simulink model "task4_simulink"  (R2026a)
settings: Solver=VariableStepAuto  StopTime=2
values from neighbouring files (symbols this model uses):
  K = place(A, B, desired_poles)    [task3.m]    (also in task4.m; task5.m; task5_original.m)
  x0 = initial_conditions(i,:)'    [task4.m]    (also in task5.m = [0; task5_original.m = [0)
settings Model: Creator=DELL  LastModifiedBy=DELL

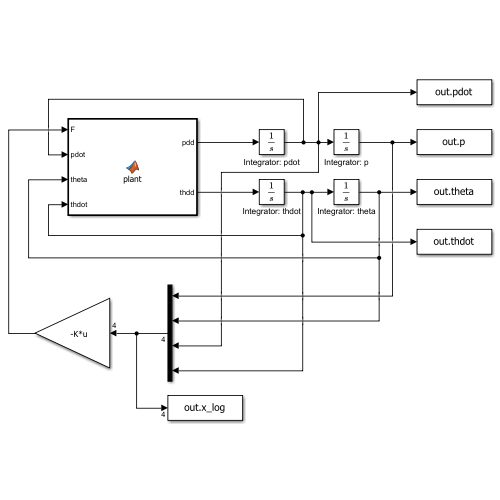
[thumbnail: Simulink's stored preview of the top-level diagram]
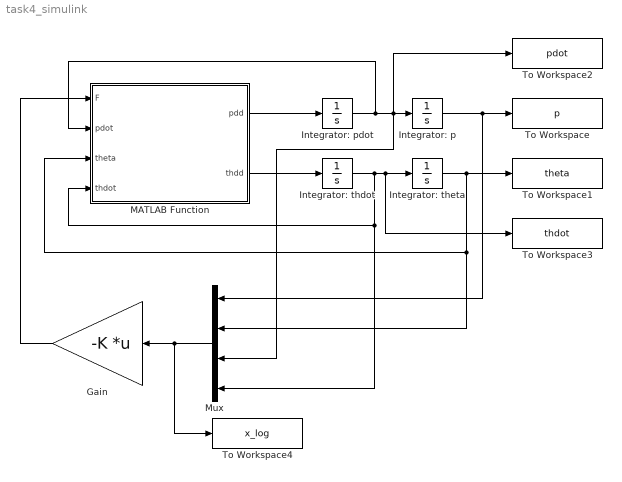
== system task4_simulink ==
  Gain : Gain  Gain=-K  Multiplication=Matrix(K*u)
  Integrator: p : Integrator  InitialCondition=x0(1)
  Integrator: pdot : Integrator  InitialCondition=x0(3)
  Integrator: thdot : Integrator  InitialCondition=x0(4)
  Integrator: theta : Integrator  InitialCondition=x0(2)
  MATLAB Function : MATLAB Function  TreatAsAtomicUnit=on
  Mux : Mux
  To Workspace : ToWorkspace  VariableName=p  SaveFormat=Timeseries  SampleTime=0.01
  To Workspace1 : ToWorkspace  VariableName=theta  SaveFormat=Timeseries  SampleTime=0.01
  To Workspace2 : ToWorkspace  VariableName=pdot  SaveFormat=Timeseries  SampleTime=-1
  To Workspace3 : ToWorkspace  VariableName=thdot  SaveFormat=Timeseries  SampleTime=-1
  To Workspace4 : ToWorkspace  VariableName=x_log  SaveFormat=Timeseries  SampleTime=0.01
  wires:
  MATLAB Function/1(pdd) -> Integrator: pdot/1
  MATLAB Function/2(thdd) -> Integrator: thdot/1
  Integrator: pdot/1 -> MATLAB Function/2(pdot), To Workspace2/1, Integrator: p/1, Mux/3
  Integrator: thdot/1 -> Mux/4, MATLAB Function/4(thdot), To Workspace3/1, Integrator: theta/1
  Integrator: theta/1 -> To Workspace1/1, Mux/2, MATLAB Function/3(theta)
  Integrator: p/1 -> Mux/1, To Workspace/1
  Mux/1 -> To Workspace4/1, Gain/1
  Gain/1 -> MATLAB Function/1(F)

== matlab function task4_simulink/MATLAB Function ==
  data: F input; pdd output; pdot input; theta input; thdot input; thdd output
function [pdd, thdd] = plant(F, pdot, theta, thdot)

M = 5;
m = 1;
l = 0.5;
c = 0.2;
g = 9.8;

pdd = ( ...
    F ...
    - c*pdot ...
    + m*g*sin(theta)*cos(theta) ...
    - m*l*sin(theta)*thdot^2 ...
    ) / (M+m-m*cos(theta)^2);

thdd = ( ...
    cos(theta)*pdd ...
    + g*sin(theta) ...
    ) / l;

end
